simulink model "posture_regulation_model"  (R2022b)
settings: Solver=VariableStepAuto  StartTime=0.0  StopTime=6  RelTol=1e-3
values from neighbouring files (symbols this model uses):
  k1 = 0.7    [posture_regulation.m]
  k2 = 0.8    [posture_regulation.m]
  k3 = 0.7    [posture_regulation.m]
  q_i = [-1 2 0]'    [posture_regulation.m]
  Ts = 0.1    [posture_regulation.m]
libraries: robotmobilelib x1
settings Model: Creator=gaetano  LastModifiedBy=gaetano

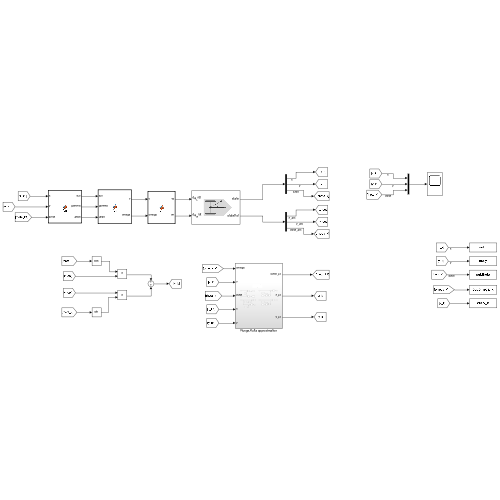
[thumbnail: Simulink's stored preview of the top-level diagram]
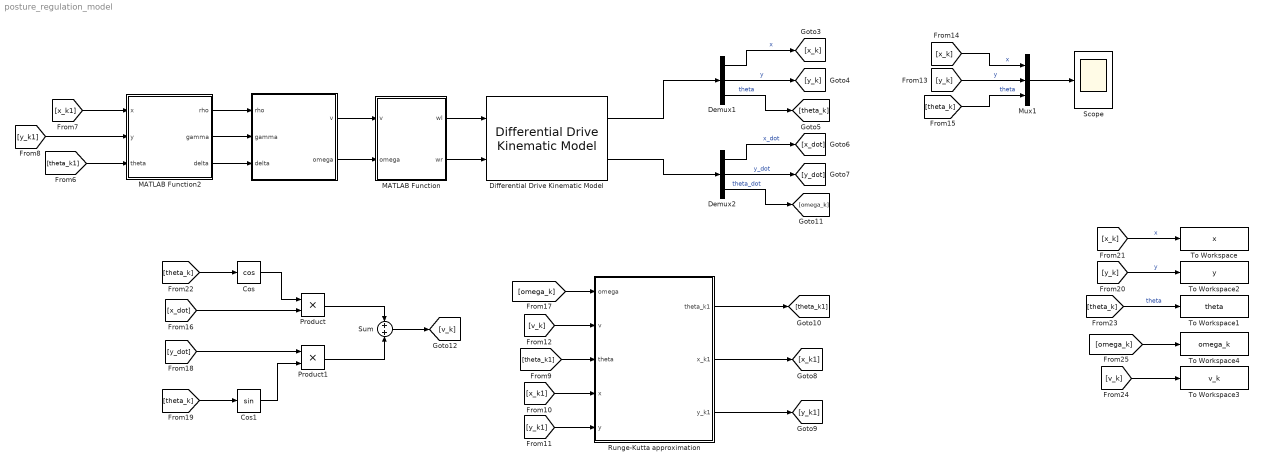
== system posture_regulation_model ==
  " " : MATLAB Function  TreatAsAtomicUnit=on
  Cos : Trigonometry  Operator=cos
  Cos1 : Trigonometry
  Demux1 : Demux  Outputs=3
  Demux2 : Demux  Outputs=3
  Differential Drive Kinematic Model : robotmobilelib/Differential Drive Kinematic Model  VehicleInputs=Wheel Speeds  WheelRadius=0.0318  WheelSpeedRange=[-inf inf]  TrackWidth=0.1232  InitialState=q_i  SimulateUsing=Interpreted execution
  MATLAB Function : MATLAB Function  TreatAsAtomicUnit=on
  MATLAB Function2 : MATLAB Function  TreatAsAtomicUnit=on
  Mux1 : Mux  Inputs=3
  Product : Product
  Product1 : Product
  Runge-Kutta approximation : Subsystem
  Scope : Scope
  Sum : Sum  Inputs=+|+
  To Workspace : ToWorkspace  VariableName=x  SaveFormat=Timeseries  SampleTime=-1
  To Workspace1 : ToWorkspace  VariableName=theta  SaveFormat=Timeseries  SampleTime=-1
  To Workspace2 : ToWorkspace  VariableName=y  SaveFormat=Timeseries  SampleTime=-1
  To Workspace3 : ToWorkspace  VariableName=v_k  SaveFormat=Timeseries  SampleTime=-1
  To Workspace4 : ToWorkspace  VariableName=omega_k  SaveFormat=Timeseries  SampleTime=-1
  wires:
  " "/2(omega) -> MATLAB Function/2(omega)
  " "/1(v) -> MATLAB Function/1(v)
  Differential Drive Kinematic Model/1 -> Demux1/1
  MATLAB Function2/2(gamma) -> " "/2(gamma)
  Demux1/3 -> [theta_k]  "theta"
  MATLAB Function2/3(delta) -> " "/3(delta)
  Demux1/1 -> [x_k]  "x"
  MATLAB Function2/1(rho) -> " "/1(rho)
  Demux1/2 -> [y_k]  "y"
  [theta_k1] -> MATLAB Function2/3(theta)
  [x_k1] -> MATLAB Function2/1(x)
  [y_k1] -> MATLAB Function2/2(y)
  Mux1/1 -> Scope/1
  [theta_k] -> Mux1/3  "theta"
  [x_k] -> Mux1/1  "x"
  [y_k] -> Mux1/2  "y"
  Differential Drive Kinematic Model/2 -> Demux2/1
  Demux2/2 -> [y_dot]  "y_dot"
  Demux2/3 -> [omega_k]  "theta_dot"
  Demux2/1 -> [x_dot]  "x_dot"
  Sum/1 -> [v_k]
  Product/1 -> Sum/1
  Product1/1 -> Sum/2
  Runge-Kutta approximation/1(theta_k1) -> [theta_k1]
  Runge-Kutta approximation/2(x_k1) -> [x_k1]
  Runge-Kutta approximation/3(y_k1) -> [y_k1]
  [theta_k1] -> Runge-Kutta approximation/3(theta)
  [x_k1] -> Runge-Kutta approximation/4(x)
  [y_k1] -> Runge-Kutta approximation/5(y)
  Cos/1 -> Product/1
  Cos1/1 -> Product1/2
  [v_k] -> Runge-Kutta approximation/2(v)
  [omega_k] -> Runge-Kutta approximation/1(omega)
  [theta_k] -> Cos1/1
  [x_dot] -> Product/2
  [y_dot] -> Product1/1
  [theta_k] -> Cos/1
  [x_k] -> To Workspace/1  "x"
  [theta_k] -> To Workspace1/1  "theta"
  [y_k] -> To Workspace2/1  "y"
  [omega_k] -> To Workspace4/1
  [v_k] -> To Workspace3/1
  MATLAB Function/1(wl) -> Differential Drive Kinematic Model/1
  MATLAB Function/2(wr) -> Differential Drive Kinematic Model/2

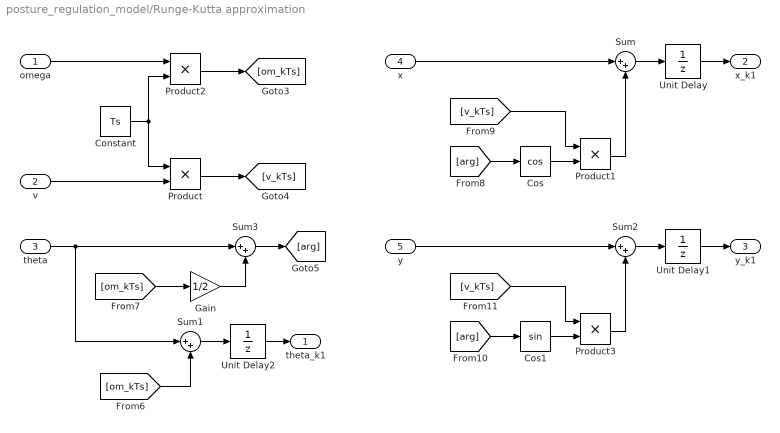
== system posture_regulation_model/Runge-Kutta approximation ==
  omega : Inport
  v : Inport  Port=2
  theta : Inport  Port=3
  x : Inport  Port=4
  y : Inport  Port=5
  Constant : Constant  Value=Ts
  Cos : Trigonometry  Operator=cos
  Cos1 : Trigonometry
  Gain : Gain  Gain=1/2
  Product{,1..3} (4 alike) : Product
  Sum{,1..3} (4 alike) : Sum  Inputs=|++
  Unit Delay : UnitDelay  InitialCondition=q_i(1)  SampleTime=Ts  HasFrameUpgradeWarning=on
  Unit Delay1 : UnitDelay  InitialCondition=q_i(2)  SampleTime=Ts  HasFrameUpgradeWarning=on
  Unit Delay2 : UnitDelay  InitialCondition=q_i(3)  SampleTime=Ts  HasFrameUpgradeWarning=on
  theta_k1 : Outport
  x_k1 : Outport  Port=2
  y_k1 : Outport  Port=3
  wires:
  Sum3/1 -> [arg]
  theta/1 -> Sum1/1, Sum3/1
  [v_kTs] -> Product3/1
  omega/1 -> Product2/1
  [om_kTs] -> Sum1/2
  [arg] -> Cos1/1
  [arg] -> Cos/1
  x/1 -> Sum/1
  Product/1 -> [v_kTs]
  y/1 -> Sum2/1
  [om_kTs] -> Gain/1
  v/1 -> Product/2
  [v_kTs] -> Product1/1
  Cos/1 -> Product1/2
  Constant/1 -> Product2/2, Product/1
  Product2/1 -> [om_kTs]
  Product1/1 -> Sum/2
  Product3/1 -> Sum2/2
  Gain/1 -> Sum3/2
  Cos1/1 -> Product3/2
  Sum1/1 -> Unit Delay2/1
  Sum2/1 -> Unit Delay1/1
  Sum/1 -> Unit Delay/1
  Unit Delay2/1 -> theta_k1/1
  Unit Delay/1 -> x_k1/1
  Unit Delay1/1 -> y_k1/1

== matlab function posture_regulation_model/MATLAB Function ==
  data: wl output; v input; omega input; wr output
function [wl, wr] = fcn(v, omega)

 raggio = 0.0318;
 interasse = 0.1232;

	wr = (2*v + omega*interasse)/(2*raggio);
	wl = (2*v - omega*interasse)/(2*raggio);

end

== matlab function posture_regulation_model/MATLAB Function2 ==
  data: x input; rho output; gamma output; y input; theta input; delta output
function [rho,gamma,delta] = fcn(x,y,theta)

rho = sqrt(x^2+y^2);

gamma = atan2(y,x) - theta + pi;
% gamma = mod(gamma + pi, 2*pi) - pi;
    while gamma > pi
        gamma = gamma - 2*pi;
    end
    
    while gamma < -pi
        gamma = gamma + 2*pi;
    end

delta = gamma + theta;

== matlab function posture_regulation_model/  ==
  data: rho input; v output; omega output; gamma input; delta input; k1 parameter; k2 parameter; k3 parameter
function [v,omega] = fcn(rho,gamma,delta, k1, k2, k3)

v = k1 * rho * cos(gamma);
omega = k2 * gamma + k1*sin(gamma)*cos(gamma)*(1+k3*delta/gamma);
